simulink model "VTS_challenge_2021"  (R2019a)
settings: Solver=ode1  StartTime=0.0  StopTime=SIMULPARAM.T_end  FixedStep=SIMULPARAM.Ts  RelTol=1e-3
undefined symbols (not defined in the file or in its folder): BAT, CHAp, EM1, EM2, EMS, MTp, RDp, Speed_control, SPEEDCONTROL
libraries: simulink x3
(part 2 of 2)

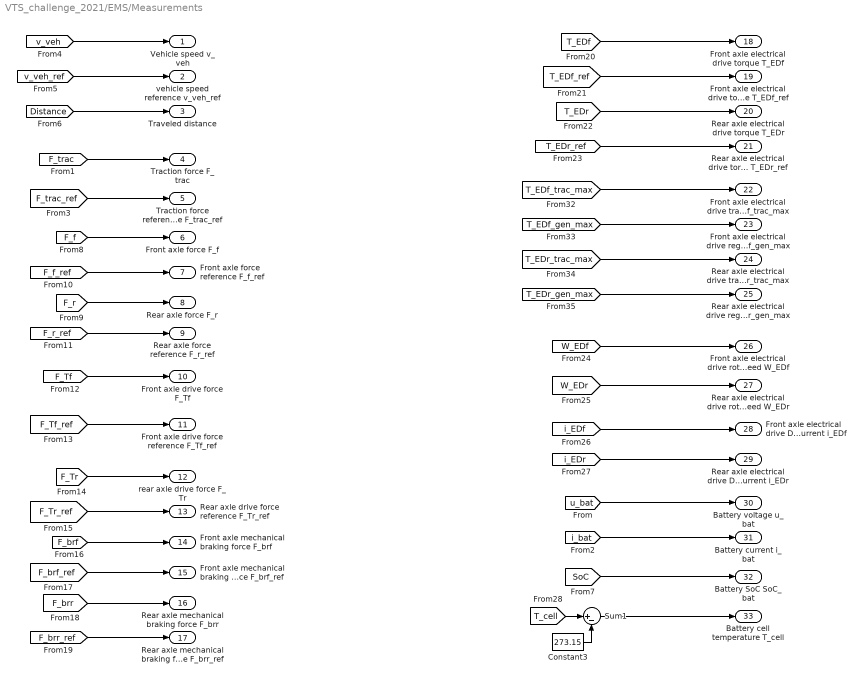
== system VTS_challenge_2021/EMS/Measurements ==
  Constant3 : Constant  Value=273.15
  Sum1 : Sum  Inputs=|+-
  Vehicle speed v_veh : Outport
  vehicle speed reference v_veh_ref : Outport  Port=2
  Traveled distance : Outport  Port=3
  Traction force F_trac : Outport  Port=4
  Traction force reference F_trac_ref : Outport  Port=5
  Front axle force F_f : Outport  Port=6
  Front axle force reference F_f_ref : Outport  Port=7
  Rear axle force F_r : Outport  Port=8
  Rear axle force reference F_r_ref : Outport  Port=9
  Front axle drive force F_Tf : Outport  Port=10
  Front axle drive force reference F_Tf_ref : Outport  Port=11
  rear axle drive force F_Tr : Outport  Port=12
  Rear axle drive force reference F_Tr_ref : Outport  Port=13
  Front axle mechanical braking force F_brf : Outport  Port=14
  Front axle mechanical braking force reference F_brf_ref : Outport  Port=15
  Rear axle mechanical braking force F_brr : Outport  Port=16
  Rear axle mechanical braking force reference F_brr_ref : Outport  Port=17
  Front axle electrical drive torque T_EDf : Outport  Port=18
  Front axle electrical drive torque reference T_EDf_ref : Outport  Port=19
  Rear axle electrical drive torque T_EDr : Outport  Port=20
  Rear axle electrical drive torque reference T_EDr_ref : Outport  Port=21
  Front axle electrical drive traction torque limitation T_EDf_trac_max : Outport  Port=22
  Front axle electrical drive regenerative torque limitation T_EDf_gen_max : Outport  Port=23
  Rear axle electrical drive traction torque limitation T_EDr_trac_max : Outport  Port=24
  Rear axle electrical drive regenerative torque limitation T_EDr_gen_max : Outport  Port=25
  Front axle electrical drive rotational speed W_EDf : Outport  Port=26
  Rear axle electrical drive rotational speed W_EDr : Outport  Port=27
  Front axle electrical drive DC bus current i_EDf : Outport  Port=28
  Rear axle electrical drive DC bus current i_EDr : Outport  Port=29
  Battery voltage u_bat : Outport  Port=30
  Battery current i_bat : Outport  Port=31
  Battery SoC SoC_bat : Outport  Port=32
  Battery cell temperature T_cell : Outport  Port=33
  wires:
  [F_trac_ref] -> Traction force reference F_trac_ref/1
  [F_brr] -> Rear axle mechanical braking force F_brr/1
  Constant3/1 -> Sum1/2
  [T_EDr_gen_max] -> Rear axle electrical drive regenerative torque limitation T_EDr_gen_max/1
  [W_EDr] -> Rear axle electrical drive rotational speed W_EDr/1
  [F_brf_ref] -> Front axle mechanical braking force reference F_brf_ref/1
  [v_veh_ref] -> vehicle speed reference v_veh_ref/1
  [T_EDr_trac_max] -> Rear axle electrical drive traction torque limitation T_EDr_trac_max/1
  [T_cell] -> Sum1/1
  [T_EDf_ref] -> Front axle electrical drive torque reference T_EDf_ref/1
  [F_brr_ref] -> Rear axle mechanical braking force reference F_brr_ref/1
  [F_r] -> Rear axle force F_r/1
  [F_r_ref] -> Rear axle force reference F_r_ref/1
  [Distance] -> Traveled distance/1
  [W_EDf] -> Front axle electrical drive rotational speed W_EDf/1
  [v_veh] -> Vehicle speed v_veh/1
  [i_EDf] -> Front axle electrical drive DC bus current i_EDf/1
  [F_Tr] -> rear axle drive force F_Tr/1
  [F_f] -> Front axle force F_f/1
  [F_Tf] -> Front axle drive force F_Tf/1
  [T_EDr] -> Rear axle electrical drive torque T_EDr/1
  [T_EDf_gen_max] -> Front axle electrical drive regenerative torque limitation T_EDf_gen_max/1
  [T_EDf_trac_max] -> Front axle electrical drive traction torque limitation T_EDf_trac_max/1
  Sum1/1 -> Battery cell temperature T_cell/1
  [SoC] -> Battery SoC SoC_bat/1
  [F_Tr_ref] -> Rear axle drive force reference F_Tr_ref/1
  [u_bat] -> Battery voltage u_bat/1
  [F_brf] -> Front axle mechanical braking force F_brf/1
  [T_EDr_ref] -> Rear axle electrical drive torque reference T_EDr_ref/1
  [i_EDr] -> Rear axle electrical drive DC bus current i_EDr/1
  [F_trac] -> Traction force F_trac/1
  [F_f_ref] -> Front axle force reference F_f_ref/1
  [F_Tf_ref] -> Front axle drive force reference F_Tf_ref/1
  [i_bat] -> Battery current i_bat/1
  [T_EDf] -> Front axle electrical drive torque T_EDf/1

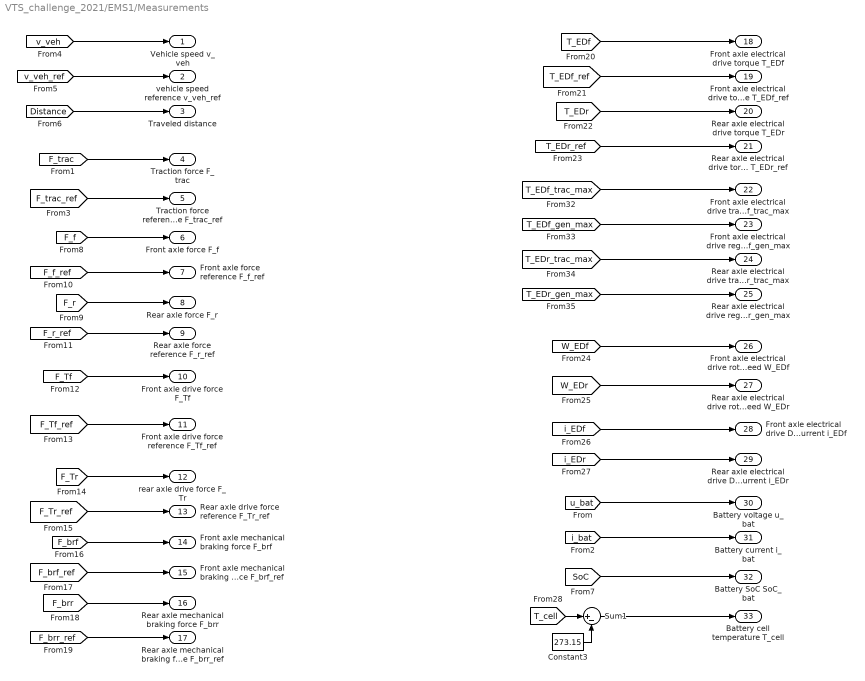
== system VTS_challenge_2021/EMS1/Measurements ==
  Constant3 : Constant  Value=273.15
  Sum1 : Sum  Inputs=|+-
  Vehicle speed v_veh : Outport
  vehicle speed reference v_veh_ref : Outport  Port=2
  Traveled distance : Outport  Port=3
  Traction force F_trac : Outport  Port=4
  Traction force reference F_trac_ref : Outport  Port=5
  Front axle force F_f : Outport  Port=6
  Front axle force reference F_f_ref : Outport  Port=7
  Rear axle force F_r : Outport  Port=8
  Rear axle force reference F_r_ref : Outport  Port=9
  Front axle drive force F_Tf : Outport  Port=10
  Front axle drive force reference F_Tf_ref : Outport  Port=11
  rear axle drive force F_Tr : Outport  Port=12
  Rear axle drive force reference F_Tr_ref : Outport  Port=13
  Front axle mechanical braking force F_brf : Outport  Port=14
  Front axle mechanical braking force reference F_brf_ref : Outport  Port=15
  Rear axle mechanical braking force F_brr : Outport  Port=16
  Rear axle mechanical braking force reference F_brr_ref : Outport  Port=17
  Front axle electrical drive torque T_EDf : Outport  Port=18
  Front axle electrical drive torque reference T_EDf_ref : Outport  Port=19
  Rear axle electrical drive torque T_EDr : Outport  Port=20
  Rear axle electrical drive torque reference T_EDr_ref : Outport  Port=21
  Front axle electrical drive traction torque limitation T_EDf_trac_max : Outport  Port=22
  Front axle electrical drive regenerative torque limitation T_EDf_gen_max : Outport  Port=23
  Rear axle electrical drive traction torque limitation T_EDr_trac_max : Outport  Port=24
  Rear axle electrical drive regenerative torque limitation T_EDr_gen_max : Outport  Port=25
  Front axle electrical drive rotational speed W_EDf : Outport  Port=26
  Rear axle electrical drive rotational speed W_EDr : Outport  Port=27
  Front axle electrical drive DC bus current i_EDf : Outport  Port=28
  Rear axle electrical drive DC bus current i_EDr : Outport  Port=29
  Battery voltage u_bat : Outport  Port=30
  Battery current i_bat : Outport  Port=31
  Battery SoC SoC_bat : Outport  Port=32
  Battery cell temperature T_cell : Outport  Port=33
  wires:
  [T_EDf] -> Front axle electrical drive torque T_EDf/1
  [i_bat] -> Battery current i_bat/1
  [F_Tf_ref] -> Front axle drive force reference F_Tf_ref/1
  [F_f_ref] -> Front axle force reference F_f_ref/1
  [F_trac] -> Traction force F_trac/1
  [i_EDr] -> Rear axle electrical drive DC bus current i_EDr/1
  [T_EDr_ref] -> Rear axle electrical drive torque reference T_EDr_ref/1
  [F_brf] -> Front axle mechanical braking force F_brf/1
  [u_bat] -> Battery voltage u_bat/1
  [F_Tr_ref] -> Rear axle drive force reference F_Tr_ref/1
  [SoC] -> Battery SoC SoC_bat/1
  Sum1/1 -> Battery cell temperature T_cell/1
  [T_EDf_trac_max] -> Front axle electrical drive traction torque limitation T_EDf_trac_max/1
  [T_EDf_gen_max] -> Front axle electrical drive regenerative torque limitation T_EDf_gen_max/1
  [T_EDr] -> Rear axle electrical drive torque T_EDr/1
  [F_Tf] -> Front axle drive force F_Tf/1
  [F_f] -> Front axle force F_f/1
  [F_Tr] -> rear axle drive force F_Tr/1
  [i_EDf] -> Front axle electrical drive DC bus current i_EDf/1
  [v_veh] -> Vehicle speed v_veh/1
  [W_EDf] -> Front axle electrical drive rotational speed W_EDf/1
  [Distance] -> Traveled distance/1
  [F_r_ref] -> Rear axle force reference F_r_ref/1
  [F_r] -> Rear axle force F_r/1
  [F_brr_ref] -> Rear axle mechanical braking force reference F_brr_ref/1
  [T_EDf_ref] -> Front axle electrical drive torque reference T_EDf_ref/1
  [T_cell] -> Sum1/1
  [T_EDr_trac_max] -> Rear axle electrical drive traction torque limitation T_EDr_trac_max/1
  [v_veh_ref] -> vehicle speed reference v_veh_ref/1
  [F_brf_ref] -> Front axle mechanical braking force reference F_brf_ref/1
  [W_EDr] -> Rear axle electrical drive rotational speed W_EDr/1
  [T_EDr_gen_max] -> Rear axle electrical drive regenerative torque limitation T_EDr_gen_max/1
  Constant3/1 -> Sum1/2
  [F_brr] -> Rear axle mechanical braking force F_brr/1
  [F_trac_ref] -> Traction force reference F_trac_ref/1

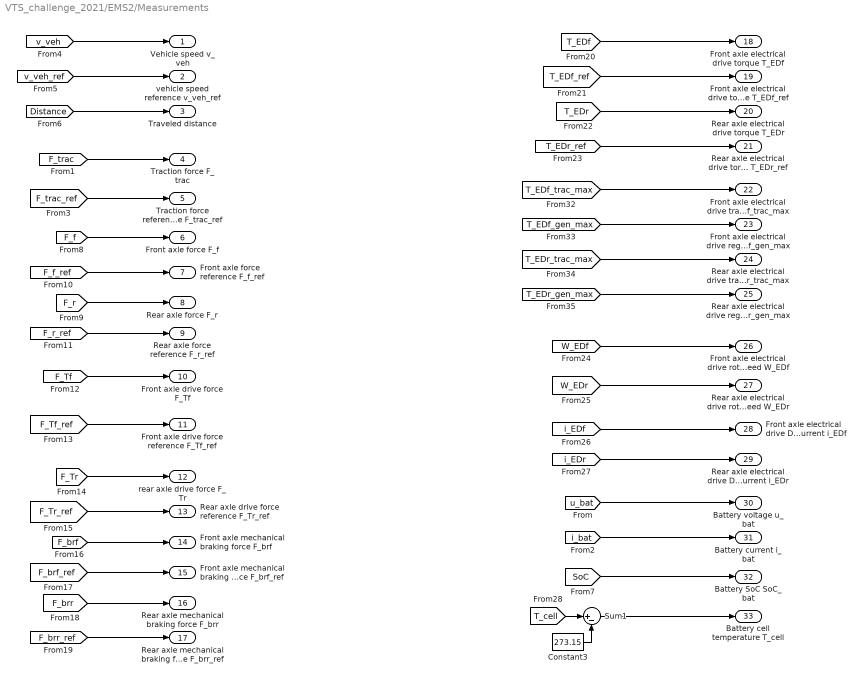
== system VTS_challenge_2021/EMS2/Measurements ==
  Constant3 : Constant  Value=273.15
  Sum1 : Sum  Inputs=|+-
  Vehicle speed v_veh : Outport
  vehicle speed reference v_veh_ref : Outport  Port=2
  Traveled distance : Outport  Port=3
  Traction force F_trac : Outport  Port=4
  Traction force reference F_trac_ref : Outport  Port=5
  Front axle force F_f : Outport  Port=6
  Front axle force reference F_f_ref : Outport  Port=7
  Rear axle force F_r : Outport  Port=8
  Rear axle force reference F_r_ref : Outport  Port=9
  Front axle drive force F_Tf : Outport  Port=10
  Front axle drive force reference F_Tf_ref : Outport  Port=11
  rear axle drive force F_Tr : Outport  Port=12
  Rear axle drive force reference F_Tr_ref : Outport  Port=13
  Front axle mechanical braking force F_brf : Outport  Port=14
  Front axle mechanical braking force reference F_brf_ref : Outport  Port=15
  Rear axle mechanical braking force F_brr : Outport  Port=16
  Rear axle mechanical braking force reference F_brr_ref : Outport  Port=17
  Front axle electrical drive torque T_EDf : Outport  Port=18
  Front axle electrical drive torque reference T_EDf_ref : Outport  Port=19
  Rear axle electrical drive torque T_EDr : Outport  Port=20
  Rear axle electrical drive torque reference T_EDr_ref : Outport  Port=21
  Front axle electrical drive traction torque limitation T_EDf_trac_max : Outport  Port=22
  Front axle electrical drive regenerative torque limitation T_EDf_gen_max : Outport  Port=23
  Rear axle electrical drive traction torque limitation T_EDr_trac_max : Outport  Port=24
  Rear axle electrical drive regenerative torque limitation T_EDr_gen_max : Outport  Port=25
  Front axle electrical drive rotational speed W_EDf : Outport  Port=26
  Rear axle electrical drive rotational speed W_EDr : Outport  Port=27
  Front axle electrical drive DC bus current i_EDf : Outport  Port=28
  Rear axle electrical drive DC bus current i_EDr : Outport  Port=29
  Battery voltage u_bat : Outport  Port=30
  Battery current i_bat : Outport  Port=31
  Battery SoC SoC_bat : Outport  Port=32
  Battery cell temperature T_cell : Outport  Port=33
  wires:
  [F_trac_ref] -> Traction force reference F_trac_ref/1
  [F_brr] -> Rear axle mechanical braking force F_brr/1
  Constant3/1 -> Sum1/2
  [T_EDr_gen_max] -> Rear axle electrical drive regenerative torque limitation T_EDr_gen_max/1
  [W_EDr] -> Rear axle electrical drive rotational speed W_EDr/1
  [F_brf_ref] -> Front axle mechanical braking force reference F_brf_ref/1
  [v_veh_ref] -> vehicle speed reference v_veh_ref/1
  [T_EDr_trac_max] -> Rear axle electrical drive traction torque limitation T_EDr_trac_max/1
  [T_cell] -> Sum1/1
  [T_EDf_ref] -> Front axle electrical drive torque reference T_EDf_ref/1
  [F_brr_ref] -> Rear axle mechanical braking force reference F_brr_ref/1
  [F_r] -> Rear axle force F_r/1
  [F_r_ref] -> Rear axle force reference F_r_ref/1
  [Distance] -> Traveled distance/1
  [W_EDf] -> Front axle electrical drive rotational speed W_EDf/1
  [v_veh] -> Vehicle speed v_veh/1
  [i_EDf] -> Front axle electrical drive DC bus current i_EDf/1
  [F_Tr] -> rear axle drive force F_Tr/1
  [F_f] -> Front axle force F_f/1
  [F_Tf] -> Front axle drive force F_Tf/1
  [T_EDr] -> Rear axle electrical drive torque T_EDr/1
  [T_EDf_gen_max] -> Front axle electrical drive regenerative torque limitation T_EDf_gen_max/1
  [T_EDf_trac_max] -> Front axle electrical drive traction torque limitation T_EDf_trac_max/1
  Sum1/1 -> Battery cell temperature T_cell/1
  [SoC] -> Battery SoC SoC_bat/1
  [F_Tr_ref] -> Rear axle drive force reference F_Tr_ref/1
  [u_bat] -> Battery voltage u_bat/1
  [F_brf] -> Front axle mechanical braking force F_brf/1
  [T_EDr_ref] -> Rear axle electrical drive torque reference T_EDr_ref/1
  [i_EDr] -> Rear axle electrical drive DC bus current i_EDr/1
  [F_trac] -> Traction force F_trac/1
  [F_f_ref] -> Front axle force reference F_f_ref/1
  [F_Tf_ref] -> Front axle drive force reference F_Tf_ref/1
  [i_bat] -> Battery current i_bat/1
  [T_EDf] -> Front axle electrical drive torque T_EDf/1

== system VTS_challenge_2021/Speed controller/IP controller ==
  v_veh_meas : Inport
  v_veh_ref : Inport  Port=2
  Gain : Gain  Gain=SPEEDCONTROL.Kp_ip
  Gain1 : Gain  Gain=SPEEDCONTROL.Ki_ip
  Integrator : Integrator
  Sum1 : Sum  Inputs=-+
  Sum3 : Sum  Inputs=+-
  F_tran_ref : Outport
  wires:
  v_veh_ref/1 -> Sum1/2
  Gain/1 -> Sum3/2
  Integrator/1 -> Gain1/1
  v_veh_meas/1 -> Sum1/1, Gain/1
  Gain1/1 -> Sum3/1
  Sum3/1 -> F_tran_ref/1
  Sum1/1 -> Integrator/1

== system VTS_challenge_2021/Speed controller/PI controller ==
  v_veh_meas : Inport
  v_veh_ref : Inport  Port=2
  Gain : Gain  Gain=SPEEDCONTROL.Kp_pi
  Gain1 : Gain  Gain=SPEEDCONTROL.Ki_pi
  Integrator : Integrator
  Sum1 : Sum  Inputs=-+
  Sum3 : Sum
  F_tran_ref : Outport
  wires:
  Sum1/1 -> Gain/1, Integrator/1
  Sum3/1 -> F_tran_ref/1
  Gain1/1 -> Sum3/1
  v_veh_meas/1 -> Sum1/1
  Integrator/1 -> Gain1/1
  Gain/1 -> Sum3/2
  v_veh_ref/1 -> Sum1/2

== matlab function VTS_challenge_2021/EMS/MATLAB Function1 ==
  data: v_curr input; k_fr output; k_brf output; k_brr output; F_req input; map_speed input; map_trq input; map_eff input; vec_T_trac input; vec_T_gen input
function [k_fr, k_brf, k_brr] = fcn(v_curr, F_req, map_speed, map_trq, map_eff, vec_T_trac, vec_T_gen)
    % INPUTS:
    %   v_curr: Vận tốc xe (m/s)
    %   F_req:  Lực kéo yêu cầu tổng (N)
    % PARAMETERS (Cài đặt trong Edit Data):
    %   map_speed:  Vector tốc độ (rad/s hoặc rpm)
    %   map_trq:    Vector mô-men (Nm)
    %   map_eff:    Ma trận hiệu suất
    %   vec_T_trac: Vector giới hạn mô-men khi KÉO (Motoring)
    %   vec_T_gen:  Vector giới hạn mô-men khi PHANH (Generating)

    % --- 1. THÔNG SỐ XE ---
    r_wheel = 0.3;      % Bán kính bánh xe (m)
    gear_ratio = 10;    % Tỷ số truyền
    
    % --- 2. CHUẨN BỊ DỮ LIỆU ---
    n_vec = map_speed(:)'; 
    t_vec = map_trq(:)';
    trac_curve = vec_T_trac(:)'; % Đường cong giới hạn Kéo
    gen_curve  = vec_T_gen(:)';  % Đường cong giới hạn Phanh
    
    % Tự động đổi đơn vị RPM -> rad/s
    if max(n_vec) > 1000
        n_vec = n_vec * (2*pi/60);
    end
    
    % Tự động đổi hiệu suất % -> 0-1
    if max(map_eff(:)) > 1
        eff_grid = map_eff / 100;
    else
        eff_grid = map_eff;
    end
    
    % --- 3. TÍNH GIỚI HẠN LỰC TẠI TỐC ĐỘ HIỆN TẠI (Dynamic Constraint) ---
    % Tính tốc độ góc trục động cơ
    w_mot = (v_curr / r_wheel) * gear_ratio;
    
    % Tra cứu giới hạn mô-men xoắn (Torque Limit) tại tốc độ này
    % Dùng interp1 để biết tại tốc độ này, động cơ chịu được tối đa bao nhiêu Nm
    T_lim_trac_val = interp1(n_vec, trac_curve, abs(w_mot), 'linear', 0);
    T_lim_gen_val  = interp1(n_vec, gen_curve,  abs(w_mot), 'linear', 0);
    
    % Quy đổi từ Mô-men (Nm) ra Lực tại bánh xe (N)
    F_lim_drive = (T_lim_trac_val * gear_ratio) / r_wheel;
    F_lim_brake = (T_lim_gen_val * gear_ratio)  / r_wheel;
    
    % Xác định giới hạn hiện hành dựa trên hành vi lái xe
    if F_req >= 0
        % Đang đạp GA (Kéo) -> Dùng giới hạn Traction
        current_F_limit = F_lim_drive;
    else
        % Đang đạp PHANH (Tái sinh) -> Dùng giới hạn Generation
        current_F_limit = F_lim_brake;
    end
    
    % Đảm bảo giới hạn tối thiểu để tránh lỗi chia cho 0
    if current_F_limit < 1; current_F_limit = 1; end

    % --- 4. TỐI ƯU HÓA PHÂN PHỐI LỰC (k) ---
    k_grid = 0 : 0.05 : 1; 
    P_min = inf;
    best_k = 0.5; 
    found_valid_k = false; % Cờ đánh dấu

    for k = k_grid
        % Tính lực yêu cầu trên từng cầu
        F_front = F_req * (1 - k);
        F_rear  = F_req * k;
        
        % --- KIỂM TRA RÀNG BUỘC (QUAN TRỌNG NHẤT) ---
        % Nếu lực phân bổ vượt quá giới hạn vật lý tại tốc độ hiện tại -> Bỏ qua
        if abs(F_front) > current_F_limit || abs(F_rear) > current_F_limit
            continue; 
        end
        
        found_valid_k = true;

        % Tính toán tiêu thụ năng lượng
        P_f = calc_power(v_curr, F_front, n_vec, t_vec, eff_grid, r_wheel, gear_ratio);
        P_r = calc_power(v_curr, F_rear,  n_vec, t_vec, eff_grid, r_wheel, gear_ratio);
        
        P_total = P_f + P_r;
        
        if P_total < P_min
            P_min = P_total;
            best_k = k;
        end
    end
    
    % --- 5. XỬ LÝ FAIL-SAFE (KHI KHÔNG TÌM ĐƯỢC K) ---
    % Trường hợp đạp thốc ga quá mạnh vượt quá tổng công suất 2 động cơ
    if ~found_valid_k
        % Nếu F_req > 2 * limit -> Chia đều để mỗi bên chịu tải ít nhất có thể
        best_k = 0.5;
    end
    
    % --- 6. OUTPUT ---
    k_fr = best_k;
    k_brf = 1; 
    k_brr = 1; 
end

% --- HÀM CON TÍNH CÔNG SUẤT ---
function P_out = calc_power(v, F, n_axis, t_axis, eff_map, r, G)
    w = (v / r) * G; 
    T = (F * r) / G;
    
    % Tra hiệu suất
    eff = interp2(n_axis, t_axis, eff_map, abs(w), abs(T), 'linear', 0.1);
    if eff < 0.01; eff = 0.01; end % Chặn dưới
    
    P_mech = T * w;
    
    % Tính công suất điện (P_elec)
    % Khi Kéo (F>0): P_elec = P_mech / eff
    % Khi Phanh (F<0): P_elec = P_mech * eff
    if F >= 0
        P_out = P_mech / eff;
    else
        P_out = P_mech * eff;
    end
end

== matlab function VTS_challenge_2021/EMS/Mới  ==
  data: v_curr input; k_fr output; k_brf output; k_brr output; F_req input; map_speed input; map_trq input; map_eff input; vec_T_trac input; vec_T_gen input
function [k_fr, k_brf, k_brr] = fcn(v_curr, F_req, map_speed, map_trq, map_eff, vec_T_trac, vec_T_gen)
    % INPUTS:
    %   v_curr: Vận tốc xe (m/s)
    %   F_req:  Lực kéo yêu cầu tổng (N)
    % PARAMETERS (Cài đặt trong Edit Data):
    %   map_speed:  Vector tốc độ (rad/s hoặc rpm)
    %   map_trq:    Vector mô-men (Nm)
    %   map_eff:    Ma trận hiệu suất
    %   vec_T_trac: Vector giới hạn mô-men khi KÉO (Motoring)
    %   vec_T_gen:  Vector giới hạn mô-men khi PHANH (Generating)

    % --- 1. THÔNG SỐ XE ---
    r_wheel = 0.3;      % Bán kính bánh xe (m)
    gear_ratio = 10;    % Tỷ số truyền
    
    % --- 2. CHUẨN BỊ DỮ LIỆU ---
    n_vec = map_speed(:)'; 
    t_vec = map_trq(:)';
    trac_curve = vec_T_trac(:)'; % Đường cong giới hạn Kéo
    gen_curve  = vec_T_gen(:)';  % Đường cong giới hạn Phanh
    
    % Tự động đổi đơn vị RPM -> rad/s
    if max(n_vec) > 1000
        n_vec = n_vec * (2*pi/60);
    end
    
    % Tự động đổi hiệu suất % -> 0-1
    if max(map_eff(:)) > 1
        eff_grid = map_eff / 100;
    else
        eff_grid = map_eff;
    end
    
    % --- 3. TÍNH GIỚI HẠN LỰC TẠI TỐC ĐỘ HIỆN TẠI (Dynamic Constraint) ---
    % Tính tốc độ góc trục động cơ
    w_mot = (v_curr / r_wheel) * gear_ratio;
    
    % Tra cứu giới hạn mô-men xoắn (Torque Limit) tại tốc độ này
    % Dùng interp1 để biết tại tốc độ này, động cơ chịu được tối đa bao nhiêu Nm
    T_lim_trac_val = interp1(n_vec, trac_curve, abs(w_mot), 'linear', 0);
    T_lim_gen_val  = interp1(n_vec, gen_curve,  abs(w_mot), 'linear', 0);
    
    % Quy đổi từ Mô-men (Nm) ra Lực tại bánh xe (N)
    F_lim_drive = (T_lim_trac_val * gear_ratio) / r_wheel;
    F_lim_brake = (T_lim_gen_val * gear_ratio)  / r_wheel;
    
    % Xác định giới hạn hiện hành dựa trên hành vi lái xe
    if F_req >= 0
        % Đang đạp GA (Kéo) -> Dùng giới hạn Traction
        current_F_limit = F_lim_drive;
    else
        % Đang đạp PHANH (Tái sinh) -> Dùng giới hạn Generation
        current_F_limit = F_lim_brake;
    end
    
    % Đảm bảo giới hạn tối thiểu để tránh lỗi chia cho 0
    if current_F_limit < 1; current_F_limit = 1; end

    % --- 4. TỐI ƯU HÓA PHÂN PHỐI LỰC (k) ---
    k_grid = 0 : 0.05 : 1; 
    P_min = inf;
    best_k = 0.5; 
    found_valid_k = false; % Cờ đánh dấu

    for k = k_grid
        % Tính lực yêu cầu trên từng cầu
        F_front = F_req * (1 - k);
        F_rear  = F_req * k;
        
        % --- KIỂM TRA RÀNG BUỘC (QUAN TRỌNG NHẤT) ---
        % Nếu lực phân bổ vượt quá giới hạn vật lý tại tốc độ hiện tại -> Bỏ qua
        if abs(F_front) > current_F_limit || abs(F_rear) > current_F_limit
            continue; 
        end
        
        found_valid_k = true;

        % Tính toán tiêu thụ năng lượng
        P_f = calc_power(v_curr, F_front, n_vec, t_vec, eff_grid, r_wheel, gear_ratio);
        P_r = calc_power(v_curr, F_rear,  n_vec, t_vec, eff_grid, r_wheel, gear_ratio);
        
        P_total = P_f + P_r;
        
        if P_total < P_min
            P_min = P_total;
            best_k = k;
        end
    end
    
    % --- 5. XỬ LÝ FAIL-SAFE (KHI KHÔNG TÌM ĐƯỢC K) ---
    % Trường hợp đạp thốc ga quá mạnh vượt quá tổng công suất 2 động cơ
    if ~found_valid_k
        % Nếu F_req > 2 * limit -> Chia đều để mỗi bên chịu tải ít nhất có thể
        best_k = 0.5;
    end
    
    % --- 6. OUTPUT ---
    k_fr = best_k;
    k_brf = 1; 
    k_brr = 1; 
end

% --- HÀM CON TÍNH CÔNG SUẤT ---
function P_out = calc_power(v, F, n_axis, t_axis, eff_map, r, G)
    w = (v / r) * G; 
    T = (F * r) / G;
    
    % Tra hiệu suất
    eff = interp2(n_axis, t_axis, eff_map, abs(w), abs(T), 'linear', 0.1);
    if eff < 0.01; eff = 0.01; end % Chặn dưới
    
    P_mech = T * w;
    
    % Tính công suất điện (P_elec)
    % Khi Kéo (F>0): P_elec = P_mech / eff
    % Khi Phanh (F<0): P_elec = P_mech * eff
    if F >= 0
        P_out = P_mech / eff;
    else
        P_out = P_mech * eff;
    end
end

== matlab function VTS_challenge_2021/EMS/Mới 1 ==
  data: v_curr input; k_fr output; k_brf output; k_brr output; F_req input; map_speed input; map_trq input; map_eff input; vec_T_trac input; vec_T_gen input
function [k_fr, k_brf, k_brr] = fcn(v_curr, F_req, map_speed, map_trq, map_eff, vec_T_trac, vec_T_gen)
    % INPUTS:
    %   v_curr: Vận tốc xe (m/s)
    %   F_req:  Lực kéo/phanh yêu cầu tổng (N)
    % PARAMETERS (Cài trong Edit Data):
    %   map_speed:  Vector tốc độ (rad/s hoặc rpm)
    %   map_trq:    Vector mô-men (Nm)
    %   map_eff:    Ma trận hiệu suất
    %   vec_T_trac: Vector giới hạn mô-men KÉO (Motoring)
    %   vec_T_gen:  Vector giới hạn mô-men PHANH (Generating)

    % --- 1. THÔNG SỐ XE (Cần khớp thực tế) ---
    r_wheel = 0.3;      % Bán kính bánh xe (m)
    gear_ratio = 10;    % Tỷ số truyền
    F_max_friction = 4000; % Lực phanh cơ tối đa mỗi trục (N) - Giả định

    % --- 2. XỬ LÝ DỮ LIỆU ĐẦU VÀO ---
    n_vec = map_speed(:)'; 
    t_vec = map_trq(:)';
    trac_curve = vec_T_trac(:)'; 
    gen_curve  = vec_T_gen(:)';  
    
    % Đổi đơn vị tốc độ (RPM -> rad/s)
    if max(n_vec) > 1000
        n_vec = n_vec * (2*pi/60);
    end
    
    % Đổi đơn vị hiệu suất (% -> 0-1)
    if max(map_eff(:)) > 1
        eff_grid = map_eff / 100;
    else
        eff_grid = map_eff;
    end
    
    % --- 3. TÍNH GIỚI HẠN ĐỘNG CƠ TẠI TỐC ĐỘ HIỆN TẠI ---
    w_mot = (v_curr / r_wheel) * gear_ratio; % Tốc độ góc trục động cơ
    
    % Tra cứu giới hạn mô-men tại tốc độ này
    T_lim_trac_val = interp1(n_vec, trac_curve, abs(w_mot), 'linear', 0);
    T_lim_gen_val  = interp1(n_vec, gen_curve,  abs(w_mot), 'linear', 0);
    
    % Quy đổi ra Lực (Force) tại bánh xe cho 1 động cơ
    F_lim_drive = (T_lim_trac_val * gear_ratio) / r_wheel;
    F_lim_regen = (T_lim_gen_val * gear_ratio)  / r_wheel;
    
    % Xác định giới hạn để kiểm tra ràng buộc
    if F_req >= 0
        current_limit = F_lim_drive; % Đang kéo
    else
        current_limit = F_lim_regen; % Đang phanh điện
    end
    
    % Tránh lỗi chia cho 0
    if current_limit < 1; current_limit = 1; end

    % --- 4. TỐI ƯU HÓA PHÂN PHỐI LỰC (k_fr) ---
    k_grid = 0 : 0.05 : 1; 
    P_min = inf;
    best_k = 0.5; 
    found_valid_k = false;

    % Chỉ chạy tối ưu hóa nếu F_req nằm trong khả năng của động cơ điện
    % Nếu F_req quá lớn (phanh gấp hoặc thốc ga), ta xử lý ở bước Fail-Safe
    total_capacity = current_limit * 2; % Giả sử 2 cầu giống nhau
    
    if abs(F_req) <= total_capacity
        for k = k_grid
            F_front = F_req * (1 - k);
            F_rear  = F_req * k;
            
            % KIỂM TRA RÀNG BUỘC (QUAN TRỌNG)
            if abs(F_front) > current_limit || abs(F_rear) > current_limit
                continue; 
            end
            
            found_valid_k = true;

            % Tính công suất tiêu thụ
            P_f = calc_power(v_curr, F_front, n_vec, t_vec, eff_grid, r_wheel, gear_ratio);
            P_r = calc_power(v_curr, F_rear,  n_vec, t_vec, eff_grid, r_wheel, gear_ratio);
            P_total = P_f + P_r;
            
            if P_total < P_min
                P_min = P_total;
                best_k = k;
            end
        end
    end
    
    % --- 5. XỬ LÝ FAIL-SAFE & PHANH CƠ KHÍ ---
    
    % Trường hợp 1: Không tìm được k (hoặc F_req quá lớn)
    if ~found_valid_k
        best_k = 0.5; % Chia đều lực điện để an toàn
    end
    
    % Gán đầu ra mô-men xoắn
    k_fr = best_k;
    
    % --- 6. TÍNH TOÁN PHANH CƠ KHÍ (k_brf, k_brr) ---
    % Logic: Nếu phanh điện (Regen) hết cỡ mà vẫn thiếu lực -> Dùng phanh cơ bù vào
    
    k_brf = 0; % Mặc định không phanh cơ
    k_brr = 0;
    
    if F_req < 0 % Đang phanh
        F_req_abs = abs(F_req);
        F_regen_total = F_lim_regen * 2; % Tổng lực phanh điện tối đa 2 cầu
        
        if F_req_abs > F_regen_total
            % Lực còn thiếu phải dùng phanh cơ
            F_friction_needed = F_req_abs - F_regen_total;
            
            % Chia lực phanh cơ (ví dụ chia đều hoặc 60/40)
            % Ở đây tính tỷ lệ trên khả năng phanh cơ tối đa (0-1)
            brake_cmd = F_friction_needed / (F_max_friction * 2);
            
            % Giới hạn max là 1
            if brake_cmd > 1; brake_cmd = 1; end
            
            k_brf = brake_cmd;
            k_brr = brake_cmd;
        end
    end
end

% --- HÀM CON ---
function P_out = calc_power(v, F, n_axis, t_axis, eff_map, r, G)
    w = (v / r) * G; 
    T = (F * r) / G;
    % Tra hiệu suất
    eff = interp2(n_axis, t_axis, eff_map, abs(w), abs(T), 'linear', 0.1);
    if eff < 0.01; eff = 0.01; end 
    
    P_mech = T * w;
    % Kéo thì chia eff, Phanh thì nhân eff
    if F >= 0
        P_out = P_mech / eff;
    else
        P_out = P_mech * eff;
    end
end

== matlab function VTS_challenge_2021/EMS1/MPC   ==
  data: F_trac_ref input; v_veh input; w_front input; w_rear input; k_fr output; k_brf output; k_brr output; SoC input; T_max_f input; T_gen_max_f input; T_max_r input; T_gen_max_r input; EM1 parameter; EM2 parameter
function [k_fr, k_brf, k_brr] = EMS_MPC_Solved(F_trac_ref, v_veh, w_front, w_rear, SoC, T_max_f, T_gen_max_f, T_max_r, T_gen_max_r, EM1, EM2)
    % --- KHAI BÁO THAM SỐ MPC ---
    k_fr = 0.5; k_brf = 0; k_brr = 0;
    R_wheel = 0.28; Gear_Ratio = 10;
    
    % Cấu hình MPC
    Horizon = 5;       % Dự báo trước 5 bước thời gian (ví dụ: 5 giây)
    dt = 1;            % Bước thời gian (seconds)
    SoC_ref = 0.6;     % Mức pin mong muốn duy trì (60%)
    Q_batt = 50000 * 3600; % Dung lượng pin (Joule) - Ví dụ: 50kWh
    Alpha = 20000;     % Trọng số phạt lệch SoC (Penalty factor)
    
    % --- 1. TÍNH TOÁN CƠ BẢN ---
    if abs(F_trac_ref) < 1e-3
        T_demand_total = 0;
    else
        T_demand_total = (F_trac_ref * R_wheel) / Gear_Ratio;
    end
    
    % --- 2. LOGIC MPC ---
    if T_demand_total >= 0
        % === CHẾ ĐỘ KÉO (TRACTION MPC) ===
        k_candidates = 0:0.1:1; % Giảm độ mịn lưới để chạy nhanh hơn (0.1 bước)
        min_Cost_Function = 1e15;
        best_k = 0.5;
        
        for i = 1:length(k_candidates)
            k_curr = k_candidates(i);
            
            % BƯỚC A: Kiểm tra ràng buộc hiện tại
            [is_valid] = CheckConstraints(k_curr, T_demand_total, T_max_f, T_max_r);
            
            if is_valid
                % BƯỚC B: Dự báo tương lai (PREDICTION)
                % Giả sử nhu cầu mô-men không đổi trong Horizon (Assumption: Constant Load)
                SoC_predicted = SoC;
                Total_P_loss = 0;
                
                for t = 1:Horizon
                    % 1. Tính tổn hao tại bước t
                    P_loss_t = CalculateCost(k_curr, T_demand_total, w_front, w_rear, EM1, EM2);
                    Total_P_loss = Total_P_loss + P_loss_t;
                    
                    % 2. Tính công suất điện tiêu thụ P_elec (P_loss + P_cơ)
                    P_mech_total = T_demand_total * ((w_front + w_rear)/2); % Ước lượng
                    P_elec = P_mech_total + P_loss_t;
                    
                    % 3. Cập nhật trạng thái SoC (Mô hình Pin)
                    % SoC_next = SoC_now - (P_elec * time) / Capacity
                    SoC_predicted = SoC_predicted - (P_elec * dt) / Q_batt;
                end
                
                % BƯỚC C: Hàm Mục Tiêu (COST FUNCTION)
                % J = Tổng tổn hao năng lượng + Phạt lệch SoC tương lai
                J = Total_P_loss + Alpha * (SoC_ref - SoC_predicted)^2;
                
                if J < min_Cost_Function
                    min_Cost_Function = J;
                    best_k = k_curr;
                end
            end
        end
        k_fr = best_k; k_brf = 0; k_brr = 0;
        
    else
        % === CHẾ ĐỘ PHANH (GIỮ NGUYÊN HOẶC LOGIC ĐƠN GIẢN) ===
        % MPC thường ít áp dụng cho phanh khẩn cấp vì an toàn là ưu tiên số 1
        T_regen_cap_f = -abs(T_gen_max_f); 
        T_regen_cap_r = -abs(T_gen_max_r);
        T_regen_total_cap = T_regen_cap_f + T_regen_cap_r;
        
        if T_demand_total > T_regen_total_cap
            k_fr = 0.6; k_brf = 1; k_brr = 1;  
        else
            k_fr = 0.6; k_brf = 0.5; k_brr = 0.5;
        end
    end
end
% --- CÁC HÀM PHỤ TRỢ (GIỮ NGUYÊN) ---
function P_loss = CalculateCost(k, T_req, w_f, w_r, Map1, Map2)
    T_f = k * T_req;
    T_r = (1 - k) * T_req;
    eff_f = get_efficiency_map(T_f, w_f, Map1); 
    eff_r = get_efficiency_map(T_r, w_r, Map2);
    if eff_f < 0.01, eff_f = 0.01; end
    if eff_r < 0.01, eff_r = 0.01; end
    P_loss = (T_f * w_f) / eff_f + (T_r * w_r) / eff_r;
end
function is_valid = CheckConstraints(k, T_req, T_max_f, T_max_r)
    T_f = k * T_req;
    T_r = (1 - k) * T_req;
    if (T_f <= T_max_f) && (T_r <= T_max_r)
        is_valid = true;
    else
        is_valid = false;
    end
end
function eff = get_efficiency_map(T, w, MapData)
    coder.extrinsic('interp2'); 
    eff = 0.85; 
    if abs(T) > 0 && abs(w) > 0
        eff = interp2(MapData.Speed, MapData.Torque, MapData.Eff, abs(w), abs(T), 'linear', 0.85);
    end
end

== matlab function VTS_challenge_2021/EMS2/MATLAB Function ==
  settings: updateMethod=DISCRETE
  data: F_trac_ref input; k_fr output; T_EDf_trac_max input; T_EDr_trac_max input; vehicle_speed input
function k_fr = PSO_kfr(F_trac_ref, T_EDf_trac_max, T_EDr_trac_max, vehicle_speed)
%#codegen
% =========================================================
% ANLPSO-based EMS for IEEE VTS 2021 (based on Scolaro et al. 2021)
% Output: k_fr (front force distribution coefficient)
% Inputs: F_trac_ref (required force), T_EDf_trac_max (front torque max), 
%         T_EDr_trac_max (rear torque max), vehicle_speed (vehicle speed [m/s] for efficiency lookup)
% =========================================================

%% ===== VEHICLE / DRIVETRAIN PARAMETERS =====
R_w = 0.30; % Wheel radius [m]
i_g = 3.0; % Gear ratio
eta_t = 0.95; % Transmission efficiency (assume constant, adjust if map-based)

%% ===== ANLPSO PARAMETERS (from Table I) =====
N_PART = 6; % Number of particles
MAX_IT = 25; % Max iterations
XI_MAX = 0.9; % Max inertia weight
XI_MIN = 0.3; % Min inertia weight
C1_MIN = 1.2;
C1_MAX = 1.8;
C = 3; % Sum of learning factors

%% ===== PENALTY COEFFICIENTS =====
GAMMA = 5000; % Torque violation penalty (large to enforce constraints)

%% ===== TORQUE → FORCE LIMITS =====
F_f_max = (T_EDf_trac_max * i_g * eta_t) / R_w;
F_r_max = (T_EDr_trac_max * i_g * eta_t) / R_w;
F_req = abs(F_trac_ref); % Use abs for bounds, but keep sign for torque

%% ===== DYNAMIC k_fr BOUNDS (Eq. 4–6) =====
margin = 0.98; % 2% safety margin
if F_req < 1e-3
    k_min = 0.0;
    k_max = 1.0;
else
    % Handle traction/braking symmetrically (article valid for both)
    F_trac_ref_max = min(F_req, F_f_max + F_r_max); % Eq. 5-6
    k_min = max(0.0, (F_r_max * margin) / F_trac_ref_max); % Adjusted Eq. 4
    k_max = min(1.0, 1.0 - (F_r_max * margin) / F_trac_ref_max);
end
% Safety
if k_min > k_max
    k_min = 0.0;
    k_max = 1.0;
end

%% ===== ANLPSO INITIALIZATION (Eq. 10-11) =====
kfr = zeros(N_PART, 1);
for i = 1:N_PART
    kfr(i) = k_min + (i-1)*(k_max - k_min)/(N_PART-1) + rand()*(k_max - k_min)/N_PART; % Eq. 10
end
v = (k_max - k_min)/4 * (2*rand(N_PART,1) - 1); % Eq. 11 (rv = 2*rand-1)

pbest = kfr;
pbest_fit = -Inf * ones(N_PART,1); % For maximization (higher is better)
gbest = kfr(1);
gbest_fit = -Inf;

%% ===== INITIAL FITNESS (maximize eta) =====
for i = 1:N_PART
    [T_f_req, T_r_req] = computeTorques(kfr(i), F_trac_ref, R_w, i_g, eta_t);
    eta_f = getEfficiencyFront(T_f_req, vehicle_speed); % Placeholder: implement based on Fig. 2
    eta_r = getEfficiencyRear(T_r_req, vehicle_speed); % Placeholder: implement based on Fig. 3
    pbest_fit(i) = fitness(eta_f, eta_r, kfr(i), T_f_req, T_r_req, T_EDf_trac_max, T_EDr_trac_max, GAMMA);
    
    if pbest_fit(i) > gbest_fit  % Maximize
        gbest_fit = pbest_fit(i);
        gbest = kfr(i);
    end
end

%% ===== ANLPSO MAIN LOOP =====
for it = 1:MAX_IT
    % Non-linear inertia weight (Eq. 13)
    xi = XI_MAX - ((it-1)/(MAX_IT-1))^0.5 * (XI_MAX - XI_MIN);
    
    % Compute adaptive learning factors (Eq. 14)
    eta_avg = mean(pbest_fit);
    eta_min = min(pbest_fit);
    c1 = zeros(N_PART,1);
    c2 = zeros(N_PART,1);
    for i = 1:N_PART
        if pbest_fit(i) < eta_avg
            c1(i) = C1_MAX - (C1_MAX - C1_MIN) * (pbest_fit(i) - eta_min) / (eta_avg - eta_min);
        else
            c1(i) = C1_MIN;
        end
        c2(i) = C - c1(i);
    end
    
    for i = 1:N_PART
        % Velocity update (Eq. 12)
        r1 = rand();
        r2 = rand();
        v(i) = xi * v(i) + c1(i)*r1*(pbest(i) - kfr(i)) + c2(i)*r2*(gbest - kfr(i));
        
        % Position update
        kfr(i) = kfr(i) + v(i);
        
        % Saturation with bounds
        kfr(i) = max(min(kfr(i), k_max), k_min);
        
        % Fitness evaluation
        [T_f_req, T_r_req] = computeTorques(kfr(i), F_trac_ref, R_w, i_g, eta_t);
        eta_f = getEfficiencyFront(T_f_req, vehicle_speed);
        eta_r = getEfficiencyRear(T_r_req, vehicle_speed);
        fit = fitness(eta_f, eta_r, kfr(i), T_f_req, T_r_req, T_EDf_trac_max, T_EDr_trac_max, GAMMA);
        
        % Personal best
        if fit > pbest_fit(i)
            pbest_fit(i) = fit;
            pbest(i) = kfr(i);
        end
        
        % Global best
        if fit > gbest_fit
            gbest_fit = fit;
            gbest = kfr(i);
        end
    end
    
    % Early stopping if converged (all particles close to gbest_fit)
    if max(pbest_fit) - min(pbest_fit) < 1e-4
        break;
    end
end

%% ===== FINAL OUTPUT =====
k_fr = min(max(gbest, k_min), k_max);

end

%% ===== FITNESS FUNCTION (maximize eta, with torque penalty) =====
function J = fitness(eta_f, eta_r, k_fr, T_f_req, T_r_req, T_f_max, T_r_max, GAMMA)
    if eta_f == 0 || eta_r == 0  % Avoid division by zero
        eta_total = 0;
    else
        eta_total = 1 / (k_fr / eta_f + (1 - k_fr) / eta_r);  % Eq. 3
    end
    penalty_torque = 0;
    if abs(T_f_req) > T_f_max
        penalty_torque = penalty_torque + GAMMA * (abs(T_f_req) - T_f_max)^2;
    end
    if abs(T_r_req) > T_r_max
        penalty_torque = penalty_torque + GAMMA * (abs(T_r_req) - T_r_max)^2;
    end
    J = eta_total - penalty_torque;  % Maximize eta, minimize penalty
end

%% ===== HELPER: Compute torques from k_fr =====
function [T_f_req, T_r_req] = computeTorques(k_fr, F_trac_ref, R_w, i_g, eta_t)
    F_f = k_fr * F_trac_ref;
    F_r = (1 - k_fr) * F_trac_ref;
    T_f_req = (F_f * R_w) / (i_g * eta_t);
    T_r_req = (F_r * R_w) / (i_g * eta_t);
end

%% ===== PLACEHOLDER: Efficiency lookup (implement based on maps Fig. 2-3) =====
function eta = getEfficiencyFront(torque, speed)
    % TODO: Implement interp2 or lookup table from Fig. 2
    % Example: eta = interp2(omega_grid, torque_grid, eta_map_front, radps_speed, torque);
    eta = 0.9;  % Placeholder, replace with actual map
end

function eta = getEfficiencyRear(torque, speed)
    % TODO: Implement interp2 from Fig. 3
    eta = 0.9;  % Placeholder
end
